simulink model "MMC_30_VSG_AD"  (R2023b)
settings: Solver=ode23t  StartTime=0.0  StopTime=2.4  RelTol=1e-3
InitFcn:
  | Rf=0.5929;
  | fn=50;
  | w0=2*pi*fn;
  | Lf=0.5*0.0135+0.01358;
  | R=0.5;
  | kf=8.5;
  | 
  | Kd=1.40543e+07;
  | lam=10; z0=0.707; zmax=1; wn0=lam/z0;
  | J0=223.613; DS0=4472.27;
  | Jmin=0.3*J0; Jmax=2.0*J0; Dmin=0.3*DS0; Dmax=2.2*DS0;
  | muJ=2906.97;
  | nu=0.15; nb=0.55; dzr=0.5; dzd=0;
  | tau=0.02; db=0.02; kpsi=14; txi=0.04;
  | Ts=0.0002; qref=0.03; dfref=0.064; dwref=0.4; dref=4;
  | lam_floor=1; scheme=1;
  | delta0=0.0712129;
  | J=J0; D=DS0;
libraries: spsIGBTDiodeLib x264, spsSeriesRLCBranchLib x140, spsVoltageMeasurementLib x132, spsCurrentMeasurementLib x6, spsSecondOrderFilterLib x3, spsThreePhaseVIMeasurementLib x2, spsDCVoltageSourceLib x2, slpidlib x2, spsGroundLib x1, spsPower3phInstantaneousLib x1, spsThreePhaseProgrammableVoltageSourceLib x1, spsThreePhaseSeriesRLCBranchLib x1
(part 5 of 5)

== system MMC_30_VSG_AD/MMC_INVERTER/MMC桥臂6/MMC子模块12 ==
  PWM : Inport
  IGBT/Diode : spsIGBTDiodeLib/IGBT//Diode  Ron=1e-3  Rs=1e5  Cs=inf  Measurements=off
  IGBT/Diode1 : spsIGBTDiodeLib/IGBT//Diode  Ron=1e-3  Rs=1e5  Cs=inf  Measurements=off
  Logical Operator : Logic  Inputs=1  AllPortsSameDT=off  OutDataTypeStr=boolean
  Logical Operator1 : Logic  Operator=NOT  AllPortsSameDT=off  OutDataTypeStr=boolean
  Series RLC Branch : spsSeriesRLCBranchLib/Series RLC Branch  LConnTagsString=__new0  RConnTagsString=__new0  BranchType=C  Resistance=1  Inductance=1e-3  SetiL0=off  InitialCurrent=0  Capacitance=C0  Setx0=on  InitialVoltage=V0  Measurements=None
  Voltage Measurement : spsVoltageMeasurementLib/Voltage Measurement  PhasorSimulation=off  OutputType=Complex  PSBequivalent=0
  V+ : PMIOPort  Side=Left
  V- : PMIOPort  Port=2  Side=Left
  VC : Outport
  wires:
  Logical Operator1/1 -> IGBT/Diode1/1
  Logical Operator/1 -> IGBT/Diode/1
  Voltage Measurement/1 -> VC/1
  PWM/1 -> Logical Operator/1, Logical Operator1/1
  connections:
  Voltage Measurement/LConn1 -- Series RLC Branch/LConn1 -- IGBT/Diode/LConn1
  V+/RConn1 -- IGBT/Diode/RConn1 -- IGBT/Diode1/LConn1
  V-/RConn1 -- IGBT/Diode1/RConn1 -- Series RLC Branch/RConn1 -- Voltage Measurement/LConn2

== system MMC_30_VSG_AD/MMC_INVERTER/MMC桥臂6/MMC子模块13 ==
  PWM : Inport
  IGBT/Diode : spsIGBTDiodeLib/IGBT//Diode  Ron=1e-3  Rs=1e5  Cs=inf  Measurements=off
  IGBT/Diode1 : spsIGBTDiodeLib/IGBT//Diode  Ron=1e-3  Rs=1e5  Cs=inf  Measurements=off
  Logical Operator : Logic  Inputs=1  AllPortsSameDT=off  OutDataTypeStr=boolean
  Logical Operator1 : Logic  Operator=NOT  AllPortsSameDT=off  OutDataTypeStr=boolean
  Series RLC Branch : spsSeriesRLCBranchLib/Series RLC Branch  LConnTagsString=__new0  RConnTagsString=__new0  BranchType=C  Resistance=1  Inductance=1e-3  SetiL0=off  InitialCurrent=0  Capacitance=C0  Setx0=on  InitialVoltage=V0  Measurements=None
  Voltage Measurement : spsVoltageMeasurementLib/Voltage Measurement  PhasorSimulation=off  OutputType=Complex  PSBequivalent=0
  V+ : PMIOPort  Side=Left
  V- : PMIOPort  Port=2  Side=Left
  VC : Outport
  wires:
  Logical Operator1/1 -> IGBT/Diode1/1
  Logical Operator/1 -> IGBT/Diode/1
  Voltage Measurement/1 -> VC/1
  PWM/1 -> Logical Operator/1, Logical Operator1/1
  connections:
  Voltage Measurement/LConn1 -- Series RLC Branch/LConn1 -- IGBT/Diode/LConn1
  V+/RConn1 -- IGBT/Diode/RConn1 -- IGBT/Diode1/LConn1
  V-/RConn1 -- IGBT/Diode1/RConn1 -- Series RLC Branch/RConn1 -- Voltage Measurement/LConn2

== system MMC_30_VSG_AD/MMC_INVERTER/MMC桥臂6/MMC子模块14 ==
  PWM : Inport
  IGBT/Diode : spsIGBTDiodeLib/IGBT//Diode  Ron=1e-3  Rs=1e5  Cs=inf  Measurements=off
  IGBT/Diode1 : spsIGBTDiodeLib/IGBT//Diode  Ron=1e-3  Rs=1e5  Cs=inf  Measurements=off
  Logical Operator : Logic  Inputs=1  AllPortsSameDT=off  OutDataTypeStr=boolean
  Logical Operator1 : Logic  Operator=NOT  AllPortsSameDT=off  OutDataTypeStr=boolean
  Series RLC Branch : spsSeriesRLCBranchLib/Series RLC Branch  LConnTagsString=__new0  RConnTagsString=__new0  BranchType=C  Resistance=1  Inductance=1e-3  SetiL0=off  InitialCurrent=0  Capacitance=C0  Setx0=on  InitialVoltage=V0  Measurements=None
  Voltage Measurement : spsVoltageMeasurementLib/Voltage Measurement  PhasorSimulation=off  OutputType=Complex  PSBequivalent=0
  V+ : PMIOPort  Side=Left
  V- : PMIOPort  Port=2  Side=Left
  VC : Outport
  wires:
  Logical Operator1/1 -> IGBT/Diode1/1
  Logical Operator/1 -> IGBT/Diode/1
  Voltage Measurement/1 -> VC/1
  PWM/1 -> Logical Operator/1, Logical Operator1/1
  connections:
  Voltage Measurement/LConn1 -- Series RLC Branch/LConn1 -- IGBT/Diode/LConn1
  V+/RConn1 -- IGBT/Diode/RConn1 -- IGBT/Diode1/LConn1
  V-/RConn1 -- IGBT/Diode1/RConn1 -- Series RLC Branch/RConn1 -- Voltage Measurement/LConn2

== system MMC_30_VSG_AD/MMC_INVERTER/MMC桥臂6/MMC子模块15 ==
  PWM : Inport
  IGBT/Diode : spsIGBTDiodeLib/IGBT//Diode  Ron=1e-3  Rs=1e5  Cs=inf  Measurements=off
  IGBT/Diode1 : spsIGBTDiodeLib/IGBT//Diode  Ron=1e-3  Rs=1e5  Cs=inf  Measurements=off
  Logical Operator : Logic  Inputs=1  AllPortsSameDT=off  OutDataTypeStr=boolean
  Logical Operator1 : Logic  Operator=NOT  AllPortsSameDT=off  OutDataTypeStr=boolean
  Series RLC Branch : spsSeriesRLCBranchLib/Series RLC Branch  LConnTagsString=__new0  RConnTagsString=__new0  BranchType=C  Resistance=1  Inductance=1e-3  SetiL0=off  InitialCurrent=0  Capacitance=C0  Setx0=on  InitialVoltage=V0  Measurements=None
  Voltage Measurement : spsVoltageMeasurementLib/Voltage Measurement  PhasorSimulation=off  OutputType=Complex  PSBequivalent=0
  V+ : PMIOPort  Side=Left
  V- : PMIOPort  Port=2  Side=Left
  VC : Outport
  wires:
  Logical Operator1/1 -> IGBT/Diode1/1
  Logical Operator/1 -> IGBT/Diode/1
  Voltage Measurement/1 -> VC/1
  PWM/1 -> Logical Operator/1, Logical Operator1/1
  connections:
  Voltage Measurement/LConn1 -- Series RLC Branch/LConn1 -- IGBT/Diode/LConn1
  V+/RConn1 -- IGBT/Diode/RConn1 -- IGBT/Diode1/LConn1
  V-/RConn1 -- IGBT/Diode1/RConn1 -- Series RLC Branch/RConn1 -- Voltage Measurement/LConn2

== system MMC_30_VSG_AD/MMC_INVERTER/MMC桥臂6/MMC子模块16 ==
  PWM : Inport
  IGBT/Diode : spsIGBTDiodeLib/IGBT//Diode  Ron=1e-3  Rs=1e5  Cs=inf  Measurements=off
  IGBT/Diode1 : spsIGBTDiodeLib/IGBT//Diode  Ron=1e-3  Rs=1e5  Cs=inf  Measurements=off
  Logical Operator : Logic  Inputs=1  AllPortsSameDT=off  OutDataTypeStr=boolean
  Logical Operator1 : Logic  Operator=NOT  AllPortsSameDT=off  OutDataTypeStr=boolean
  Series RLC Branch : spsSeriesRLCBranchLib/Series RLC Branch  LConnTagsString=__new0  RConnTagsString=__new0  BranchType=C  Resistance=1  Inductance=1e-3  SetiL0=off  InitialCurrent=0  Capacitance=C0  Setx0=on  InitialVoltage=V0  Measurements=None
  Voltage Measurement : spsVoltageMeasurementLib/Voltage Measurement  PhasorSimulation=off  OutputType=Complex  PSBequivalent=0
  V+ : PMIOPort  Side=Left
  V- : PMIOPort  Port=2  Side=Left
  VC : Outport
  wires:
  Logical Operator1/1 -> IGBT/Diode1/1
  Logical Operator/1 -> IGBT/Diode/1
  Voltage Measurement/1 -> VC/1
  PWM/1 -> Logical Operator/1, Logical Operator1/1
  connections:
  Voltage Measurement/LConn1 -- Series RLC Branch/LConn1 -- IGBT/Diode/LConn1
  V+/RConn1 -- IGBT/Diode/RConn1 -- IGBT/Diode1/LConn1
  V-/RConn1 -- IGBT/Diode1/RConn1 -- Series RLC Branch/RConn1 -- Voltage Measurement/LConn2

== system MMC_30_VSG_AD/MMC_INVERTER/MMC桥臂6/MMC子模块17 ==
  PWM : Inport
  IGBT/Diode : spsIGBTDiodeLib/IGBT//Diode  Ron=1e-3  Rs=1e5  Cs=inf  Measurements=off
  IGBT/Diode1 : spsIGBTDiodeLib/IGBT//Diode  Ron=1e-3  Rs=1e5  Cs=inf  Measurements=off
  Logical Operator : Logic  Inputs=1  AllPortsSameDT=off  OutDataTypeStr=boolean
  Logical Operator1 : Logic  Operator=NOT  AllPortsSameDT=off  OutDataTypeStr=boolean
  Series RLC Branch : spsSeriesRLCBranchLib/Series RLC Branch  LConnTagsString=__new0  RConnTagsString=__new0  BranchType=C  Resistance=1  Inductance=1e-3  SetiL0=off  InitialCurrent=0  Capacitance=C0  Setx0=on  InitialVoltage=V0  Measurements=None
  Voltage Measurement : spsVoltageMeasurementLib/Voltage Measurement  PhasorSimulation=off  OutputType=Complex  PSBequivalent=0
  V+ : PMIOPort  Side=Left
  V- : PMIOPort  Port=2  Side=Left
  VC : Outport
  wires:
  Logical Operator1/1 -> IGBT/Diode1/1
  Logical Operator/1 -> IGBT/Diode/1
  Voltage Measurement/1 -> VC/1
  PWM/1 -> Logical Operator/1, Logical Operator1/1
  connections:
  Voltage Measurement/LConn1 -- Series RLC Branch/LConn1 -- IGBT/Diode/LConn1
  V+/RConn1 -- IGBT/Diode/RConn1 -- IGBT/Diode1/LConn1
  V-/RConn1 -- IGBT/Diode1/RConn1 -- Series RLC Branch/RConn1 -- Voltage Measurement/LConn2

== system MMC_30_VSG_AD/MMC_INVERTER/MMC桥臂6/MMC子模块18 ==
  PWM : Inport
  IGBT/Diode : spsIGBTDiodeLib/IGBT//Diode  Ron=1e-3  Rs=1e5  Cs=inf  Measurements=off
  IGBT/Diode1 : spsIGBTDiodeLib/IGBT//Diode  Ron=1e-3  Rs=1e5  Cs=inf  Measurements=off
  Logical Operator : Logic  Inputs=1  AllPortsSameDT=off  OutDataTypeStr=boolean
  Logical Operator1 : Logic  Operator=NOT  AllPortsSameDT=off  OutDataTypeStr=boolean
  Series RLC Branch : spsSeriesRLCBranchLib/Series RLC Branch  LConnTagsString=__new0  RConnTagsString=__new0  BranchType=C  Resistance=1  Inductance=1e-3  SetiL0=off  InitialCurrent=0  Capacitance=C0  Setx0=on  InitialVoltage=V0  Measurements=None
  Voltage Measurement : spsVoltageMeasurementLib/Voltage Measurement  PhasorSimulation=off  OutputType=Complex  PSBequivalent=0
  V+ : PMIOPort  Side=Left
  V- : PMIOPort  Port=2  Side=Left
  VC : Outport
  wires:
  Logical Operator1/1 -> IGBT/Diode1/1
  Logical Operator/1 -> IGBT/Diode/1
  Voltage Measurement/1 -> VC/1
  PWM/1 -> Logical Operator/1, Logical Operator1/1
  connections:
  Voltage Measurement/LConn1 -- Series RLC Branch/LConn1 -- IGBT/Diode/LConn1
  V+/RConn1 -- IGBT/Diode/RConn1 -- IGBT/Diode1/LConn1
  V-/RConn1 -- IGBT/Diode1/RConn1 -- Series RLC Branch/RConn1 -- Voltage Measurement/LConn2

== system MMC_30_VSG_AD/MMC_INVERTER/MMC桥臂6/MMC子模块19 ==
  PWM : Inport
  IGBT/Diode : spsIGBTDiodeLib/IGBT//Diode  Ron=1e-3  Rs=1e5  Cs=inf  Measurements=off
  IGBT/Diode1 : spsIGBTDiodeLib/IGBT//Diode  Ron=1e-3  Rs=1e5  Cs=inf  Measurements=off
  Logical Operator : Logic  Inputs=1  AllPortsSameDT=off  OutDataTypeStr=boolean
  Logical Operator1 : Logic  Operator=NOT  AllPortsSameDT=off  OutDataTypeStr=boolean
  Series RLC Branch : spsSeriesRLCBranchLib/Series RLC Branch  LConnTagsString=__new0  RConnTagsString=__new0  BranchType=C  Resistance=1  Inductance=1e-3  SetiL0=off  InitialCurrent=0  Capacitance=C0  Setx0=on  InitialVoltage=V0  Measurements=None
  Voltage Measurement : spsVoltageMeasurementLib/Voltage Measurement  PhasorSimulation=off  OutputType=Complex  PSBequivalent=0
  V+ : PMIOPort  Side=Left
  V- : PMIOPort  Port=2  Side=Left
  VC : Outport
  wires:
  Logical Operator1/1 -> IGBT/Diode1/1
  Logical Operator/1 -> IGBT/Diode/1
  Voltage Measurement/1 -> VC/1
  PWM/1 -> Logical Operator/1, Logical Operator1/1
  connections:
  Voltage Measurement/LConn1 -- Series RLC Branch/LConn1 -- IGBT/Diode/LConn1
  V+/RConn1 -- IGBT/Diode/RConn1 -- IGBT/Diode1/LConn1
  V-/RConn1 -- IGBT/Diode1/RConn1 -- Series RLC Branch/RConn1 -- Voltage Measurement/LConn2

== system MMC_30_VSG_AD/MMC_INVERTER/MMC桥臂6/MMC子模块2 ==
  PWM : Inport
  IGBT/Diode : spsIGBTDiodeLib/IGBT//Diode  Ron=1e-3  Rs=1e5  Cs=inf  Measurements=off
  IGBT/Diode1 : spsIGBTDiodeLib/IGBT//Diode  Ron=1e-3  Rs=1e5  Cs=inf  Measurements=off
  Logical Operator : Logic  Inputs=1  AllPortsSameDT=off  OutDataTypeStr=boolean
  Logical Operator1 : Logic  Operator=NOT  AllPortsSameDT=off  OutDataTypeStr=boolean
  Series RLC Branch : spsSeriesRLCBranchLib/Series RLC Branch  LConnTagsString=__new0  RConnTagsString=__new0  BranchType=C  Resistance=1  Inductance=1e-3  SetiL0=off  InitialCurrent=0  Capacitance=C0  Setx0=on  InitialVoltage=V0  Measurements=None
  Voltage Measurement : spsVoltageMeasurementLib/Voltage Measurement  PhasorSimulation=off  OutputType=Complex  PSBequivalent=0
  V+ : PMIOPort  Side=Left
  V- : PMIOPort  Port=2  Side=Left
  VC : Outport
  wires:
  Logical Operator1/1 -> IGBT/Diode1/1
  Logical Operator/1 -> IGBT/Diode/1
  Voltage Measurement/1 -> VC/1
  PWM/1 -> Logical Operator/1, Logical Operator1/1
  connections:
  Voltage Measurement/LConn1 -- Series RLC Branch/LConn1 -- IGBT/Diode/LConn1
  V+/RConn1 -- IGBT/Diode/RConn1 -- IGBT/Diode1/LConn1
  V-/RConn1 -- IGBT/Diode1/RConn1 -- Series RLC Branch/RConn1 -- Voltage Measurement/LConn2

== system MMC_30_VSG_AD/MMC_INVERTER/MMC桥臂6/MMC子模块20 ==
  PWM : Inport
  IGBT/Diode : spsIGBTDiodeLib/IGBT//Diode  Ron=1e-3  Rs=1e5  Cs=inf  Measurements=off
  IGBT/Diode1 : spsIGBTDiodeLib/IGBT//Diode  Ron=1e-3  Rs=1e5  Cs=inf  Measurements=off
  Logical Operator : Logic  Inputs=1  AllPortsSameDT=off  OutDataTypeStr=boolean
  Logical Operator1 : Logic  Operator=NOT  AllPortsSameDT=off  OutDataTypeStr=boolean
  Series RLC Branch : spsSeriesRLCBranchLib/Series RLC Branch  LConnTagsString=__new0  RConnTagsString=__new0  BranchType=C  Resistance=1  Inductance=1e-3  SetiL0=off  InitialCurrent=0  Capacitance=C0  Setx0=on  InitialVoltage=V0  Measurements=None
  Voltage Measurement : spsVoltageMeasurementLib/Voltage Measurement  PhasorSimulation=off  OutputType=Complex  PSBequivalent=0
  V+ : PMIOPort  Side=Left
  V- : PMIOPort  Port=2  Side=Left
  VC : Outport
  wires:
  Logical Operator1/1 -> IGBT/Diode1/1
  Logical Operator/1 -> IGBT/Diode/1
  Voltage Measurement/1 -> VC/1
  PWM/1 -> Logical Operator/1, Logical Operator1/1
  connections:
  Voltage Measurement/LConn1 -- Series RLC Branch/LConn1 -- IGBT/Diode/LConn1
  V+/RConn1 -- IGBT/Diode/RConn1 -- IGBT/Diode1/LConn1
  V-/RConn1 -- IGBT/Diode1/RConn1 -- Series RLC Branch/RConn1 -- Voltage Measurement/LConn2

== system MMC_30_VSG_AD/MMC_INVERTER/MMC桥臂6/MMC子模块21 ==
  PWM : Inport
  IGBT/Diode : spsIGBTDiodeLib/IGBT//Diode  Ron=1e-3  Rs=1e5  Cs=inf  Measurements=off
  IGBT/Diode1 : spsIGBTDiodeLib/IGBT//Diode  Ron=1e-3  Rs=1e5  Cs=inf  Measurements=off
  Logical Operator : Logic  Inputs=1  AllPortsSameDT=off  OutDataTypeStr=boolean
  Logical Operator1 : Logic  Operator=NOT  AllPortsSameDT=off  OutDataTypeStr=boolean
  Series RLC Branch : spsSeriesRLCBranchLib/Series RLC Branch  LConnTagsString=__new0  RConnTagsString=__new0  BranchType=C  Resistance=1  Inductance=1e-3  SetiL0=off  InitialCurrent=0  Capacitance=C0  Setx0=on  InitialVoltage=V0  Measurements=None
  Voltage Measurement : spsVoltageMeasurementLib/Voltage Measurement  PhasorSimulation=off  OutputType=Complex  PSBequivalent=0
  V+ : PMIOPort  Side=Left
  V- : PMIOPort  Port=2  Side=Left
  VC : Outport
  wires:
  Logical Operator1/1 -> IGBT/Diode1/1
  Logical Operator/1 -> IGBT/Diode/1
  Voltage Measurement/1 -> VC/1
  PWM/1 -> Logical Operator/1, Logical Operator1/1
  connections:
  Voltage Measurement/LConn1 -- Series RLC Branch/LConn1 -- IGBT/Diode/LConn1
  V+/RConn1 -- IGBT/Diode/RConn1 -- IGBT/Diode1/LConn1
  V-/RConn1 -- IGBT/Diode1/RConn1 -- Series RLC Branch/RConn1 -- Voltage Measurement/LConn2

== system MMC_30_VSG_AD/MMC_INVERTER/MMC桥臂6/MMC子模块3 ==
  PWM : Inport
  IGBT/Diode : spsIGBTDiodeLib/IGBT//Diode  Ron=1e-3  Rs=1e5  Cs=inf  Measurements=off
  IGBT/Diode1 : spsIGBTDiodeLib/IGBT//Diode  Ron=1e-3  Rs=1e5  Cs=inf  Measurements=off
  Logical Operator : Logic  Inputs=1  AllPortsSameDT=off  OutDataTypeStr=boolean
  Logical Operator1 : Logic  Operator=NOT  AllPortsSameDT=off  OutDataTypeStr=boolean
  Series RLC Branch : spsSeriesRLCBranchLib/Series RLC Branch  LConnTagsString=__new0  RConnTagsString=__new0  BranchType=C  Resistance=1  Inductance=1e-3  SetiL0=off  InitialCurrent=0  Capacitance=C0  Setx0=on  InitialVoltage=V0  Measurements=None
  Voltage Measurement : spsVoltageMeasurementLib/Voltage Measurement  PhasorSimulation=off  OutputType=Complex  PSBequivalent=0
  V+ : PMIOPort  Side=Left
  V- : PMIOPort  Port=2  Side=Left
  VC : Outport
  wires:
  Logical Operator1/1 -> IGBT/Diode1/1
  Logical Operator/1 -> IGBT/Diode/1
  Voltage Measurement/1 -> VC/1
  PWM/1 -> Logical Operator/1, Logical Operator1/1
  connections:
  Voltage Measurement/LConn1 -- Series RLC Branch/LConn1 -- IGBT/Diode/LConn1
  V+/RConn1 -- IGBT/Diode/RConn1 -- IGBT/Diode1/LConn1
  V-/RConn1 -- IGBT/Diode1/RConn1 -- Series RLC Branch/RConn1 -- Voltage Measurement/LConn2

== system MMC_30_VSG_AD/MMC_INVERTER/MMC桥臂6/MMC子模块4 ==
  PWM : Inport
  IGBT/Diode : spsIGBTDiodeLib/IGBT//Diode  Ron=1e-3  Rs=1e5  Cs=inf  Measurements=off
  IGBT/Diode1 : spsIGBTDiodeLib/IGBT//Diode  Ron=1e-3  Rs=1e5  Cs=inf  Measurements=off
  Logical Operator : Logic  Inputs=1  AllPortsSameDT=off  OutDataTypeStr=boolean
  Logical Operator1 : Logic  Operator=NOT  AllPortsSameDT=off  OutDataTypeStr=boolean
  Series RLC Branch : spsSeriesRLCBranchLib/Series RLC Branch  LConnTagsString=__new0  RConnTagsString=__new0  BranchType=C  Resistance=1  Inductance=1e-3  SetiL0=off  InitialCurrent=0  Capacitance=C0  Setx0=on  InitialVoltage=V0  Measurements=None
  Voltage Measurement : spsVoltageMeasurementLib/Voltage Measurement  PhasorSimulation=off  OutputType=Complex  PSBequivalent=0
  V+ : PMIOPort  Side=Left
  V- : PMIOPort  Port=2  Side=Left
  VC : Outport
  wires:
  Logical Operator1/1 -> IGBT/Diode1/1
  Logical Operator/1 -> IGBT/Diode/1
  Voltage Measurement/1 -> VC/1
  PWM/1 -> Logical Operator/1, Logical Operator1/1
  connections:
  Voltage Measurement/LConn1 -- Series RLC Branch/LConn1 -- IGBT/Diode/LConn1
  V+/RConn1 -- IGBT/Diode/RConn1 -- IGBT/Diode1/LConn1
  V-/RConn1 -- IGBT/Diode1/RConn1 -- Series RLC Branch/RConn1 -- Voltage Measurement/LConn2

== system MMC_30_VSG_AD/MMC_INVERTER/MMC桥臂6/MMC子模块5 ==
  PWM : Inport
  IGBT/Diode : spsIGBTDiodeLib/IGBT//Diode  Ron=1e-3  Rs=1e5  Cs=inf  Measurements=off
  IGBT/Diode1 : spsIGBTDiodeLib/IGBT//Diode  Ron=1e-3  Rs=1e5  Cs=inf  Measurements=off
  Logical Operator : Logic  Inputs=1  AllPortsSameDT=off  OutDataTypeStr=boolean
  Logical Operator1 : Logic  Operator=NOT  AllPortsSameDT=off  OutDataTypeStr=boolean
  Series RLC Branch : spsSeriesRLCBranchLib/Series RLC Branch  LConnTagsString=__new0  RConnTagsString=__new0  BranchType=C  Resistance=1  Inductance=1e-3  SetiL0=off  InitialCurrent=0  Capacitance=C0  Setx0=on  InitialVoltage=V0  Measurements=None
  Voltage Measurement : spsVoltageMeasurementLib/Voltage Measurement  PhasorSimulation=off  OutputType=Complex  PSBequivalent=0
  V+ : PMIOPort  Side=Left
  V- : PMIOPort  Port=2  Side=Left
  VC : Outport
  wires:
  Logical Operator1/1 -> IGBT/Diode1/1
  Logical Operator/1 -> IGBT/Diode/1
  Voltage Measurement/1 -> VC/1
  PWM/1 -> Logical Operator/1, Logical Operator1/1
  connections:
  Voltage Measurement/LConn1 -- Series RLC Branch/LConn1 -- IGBT/Diode/LConn1
  V+/RConn1 -- IGBT/Diode/RConn1 -- IGBT/Diode1/LConn1
  V-/RConn1 -- IGBT/Diode1/RConn1 -- Series RLC Branch/RConn1 -- Voltage Measurement/LConn2

== system MMC_30_VSG_AD/MMC_INVERTER/MMC桥臂6/MMC子模块6 ==
  PWM : Inport
  IGBT/Diode : spsIGBTDiodeLib/IGBT//Diode  Ron=1e-3  Rs=1e5  Cs=inf  Measurements=off
  IGBT/Diode1 : spsIGBTDiodeLib/IGBT//Diode  Ron=1e-3  Rs=1e5  Cs=inf  Measurements=off
  Logical Operator : Logic  Inputs=1  AllPortsSameDT=off  OutDataTypeStr=boolean
  Logical Operator1 : Logic  Operator=NOT  AllPortsSameDT=off  OutDataTypeStr=boolean
  Series RLC Branch : spsSeriesRLCBranchLib/Series RLC Branch  LConnTagsString=__new0  RConnTagsString=__new0  BranchType=C  Resistance=1  Inductance=1e-3  SetiL0=off  InitialCurrent=0  Capacitance=C0  Setx0=on  InitialVoltage=V0  Measurements=None
  Voltage Measurement : spsVoltageMeasurementLib/Voltage Measurement  PhasorSimulation=off  OutputType=Complex  PSBequivalent=0
  V+ : PMIOPort  Side=Left
  V- : PMIOPort  Port=2  Side=Left
  VC : Outport
  wires:
  Logical Operator1/1 -> IGBT/Diode1/1
  Logical Operator/1 -> IGBT/Diode/1
  Voltage Measurement/1 -> VC/1
  PWM/1 -> Logical Operator/1, Logical Operator1/1
  connections:
  Voltage Measurement/LConn1 -- Series RLC Branch/LConn1 -- IGBT/Diode/LConn1
  V+/RConn1 -- IGBT/Diode/RConn1 -- IGBT/Diode1/LConn1
  V-/RConn1 -- IGBT/Diode1/RConn1 -- Series RLC Branch/RConn1 -- Voltage Measurement/LConn2

== system MMC_30_VSG_AD/MMC_INVERTER/MMC桥臂6/MMC子模块7 ==
  PWM : Inport
  IGBT/Diode : spsIGBTDiodeLib/IGBT//Diode  Ron=1e-3  Rs=1e5  Cs=inf  Measurements=off
  IGBT/Diode1 : spsIGBTDiodeLib/IGBT//Diode  Ron=1e-3  Rs=1e5  Cs=inf  Measurements=off
  Logical Operator : Logic  Inputs=1  AllPortsSameDT=off  OutDataTypeStr=boolean
  Logical Operator1 : Logic  Operator=NOT  AllPortsSameDT=off  OutDataTypeStr=boolean
  Series RLC Branch : spsSeriesRLCBranchLib/Series RLC Branch  LConnTagsString=__new0  RConnTagsString=__new0  BranchType=C  Resistance=1  Inductance=1e-3  SetiL0=off  InitialCurrent=0  Capacitance=C0  Setx0=on  InitialVoltage=V0  Measurements=None
  Voltage Measurement : spsVoltageMeasurementLib/Voltage Measurement  PhasorSimulation=off  OutputType=Complex  PSBequivalent=0
  V+ : PMIOPort  Side=Left
  V- : PMIOPort  Port=2  Side=Left
  VC : Outport
  wires:
  Logical Operator1/1 -> IGBT/Diode1/1
  Logical Operator/1 -> IGBT/Diode/1
  Voltage Measurement/1 -> VC/1
  PWM/1 -> Logical Operator/1, Logical Operator1/1
  connections:
  Voltage Measurement/LConn1 -- Series RLC Branch/LConn1 -- IGBT/Diode/LConn1
  V+/RConn1 -- IGBT/Diode/RConn1 -- IGBT/Diode1/LConn1
  V-/RConn1 -- IGBT/Diode1/RConn1 -- Series RLC Branch/RConn1 -- Voltage Measurement/LConn2

== system MMC_30_VSG_AD/MMC_INVERTER/MMC桥臂6/MMC子模块8 ==
  PWM : Inport
  IGBT/Diode : spsIGBTDiodeLib/IGBT//Diode  Ron=1e-3  Rs=1e5  Cs=inf  Measurements=off
  IGBT/Diode1 : spsIGBTDiodeLib/IGBT//Diode  Ron=1e-3  Rs=1e5  Cs=inf  Measurements=off
  Logical Operator : Logic  Inputs=1  AllPortsSameDT=off  OutDataTypeStr=boolean
  Logical Operator1 : Logic  Operator=NOT  AllPortsSameDT=off  OutDataTypeStr=boolean
  Series RLC Branch : spsSeriesRLCBranchLib/Series RLC Branch  LConnTagsString=__new0  RConnTagsString=__new0  BranchType=C  Resistance=1  Inductance=1e-3  SetiL0=off  InitialCurrent=0  Capacitance=C0  Setx0=on  InitialVoltage=V0  Measurements=None
  Voltage Measurement : spsVoltageMeasurementLib/Voltage Measurement  PhasorSimulation=off  OutputType=Complex  PSBequivalent=0
  V+ : PMIOPort  Side=Left
  V- : PMIOPort  Port=2  Side=Left
  VC : Outport
  wires:
  Logical Operator1/1 -> IGBT/Diode1/1
  Logical Operator/1 -> IGBT/Diode/1
  Voltage Measurement/1 -> VC/1
  PWM/1 -> Logical Operator/1, Logical Operator1/1
  connections:
  Voltage Measurement/LConn1 -- Series RLC Branch/LConn1 -- IGBT/Diode/LConn1
  V+/RConn1 -- IGBT/Diode/RConn1 -- IGBT/Diode1/LConn1
  V-/RConn1 -- IGBT/Diode1/RConn1 -- Series RLC Branch/RConn1 -- Voltage Measurement/LConn2

== system MMC_30_VSG_AD/MMC_INVERTER/MMC桥臂6/MMC子模块9 ==
  PWM : Inport
  IGBT/Diode : spsIGBTDiodeLib/IGBT//Diode  Ron=1e-3  Rs=1e5  Cs=inf  Measurements=off
  IGBT/Diode1 : spsIGBTDiodeLib/IGBT//Diode  Ron=1e-3  Rs=1e5  Cs=inf  Measurements=off
  Logical Operator : Logic  Inputs=1  AllPortsSameDT=off  OutDataTypeStr=boolean
  Logical Operator1 : Logic  Operator=NOT  AllPortsSameDT=off  OutDataTypeStr=boolean
  Series RLC Branch : spsSeriesRLCBranchLib/Series RLC Branch  LConnTagsString=__new0  RConnTagsString=__new0  BranchType=C  Resistance=1  Inductance=1e-3  SetiL0=off  InitialCurrent=0  Capacitance=C0  Setx0=on  InitialVoltage=V0  Measurements=None
  Voltage Measurement : spsVoltageMeasurementLib/Voltage Measurement  PhasorSimulation=off  OutputType=Complex  PSBequivalent=0
  V+ : PMIOPort  Side=Left
  V- : PMIOPort  Port=2  Side=Left
  VC : Outport
  wires:
  Logical Operator1/1 -> IGBT/Diode1/1
  Logical Operator/1 -> IGBT/Diode/1
  Voltage Measurement/1 -> VC/1
  PWM/1 -> Logical Operator/1, Logical Operator1/1
  connections:
  Voltage Measurement/LConn1 -- Series RLC Branch/LConn1 -- IGBT/Diode/LConn1
  V+/RConn1 -- IGBT/Diode/RConn1 -- IGBT/Diode1/LConn1
  V-/RConn1 -- IGBT/Diode1/RConn1 -- Series RLC Branch/RConn1 -- Voltage Measurement/LConn2

== matlab function MMC_30_VSG_AD/VSG控制/VSG有功控制-频率调节-一次调频/adap_law ==
  data: dw input; Jm output; Dm output; wn_o output; z_o output; xi_o output; Ts parameter; tau parameter; qref parameter; txi parameter; kpsi parameter; db parameter; wn0 parameter; nu parameter; nb parameter; z0 parameter; dzd parameter; dzr parameter; lam parameter; zmax parameter; Kd parameter; lam_floor parameter; scheme parameter; Jmin parameter; Jmax parameter; Dmin parameter; Dmax parameter; w0 parameter
function [Jm, Dm, wn_o, z_o, xi_o] = adap_law(dw, Ts, tau, qref, txi, kpsi, db, wn0, nu, nb, z0, dzd, dzr, lam, zmax, Kd, lam_floor, scheme, Jmin, Jmax, Dmin, Dmax, w0)





persistent dwf dwp ddwf xf first


if isempty(first)


    dwf = 0; dwp = 0; ddwf = 0; xf = 0; first = 1;


end


a = Ts/(tau + Ts);


dwf = dwf + a*(dw - dwf);               


d1  = (dwf - dwp)/Ts;


dwp = dwf;


ddwf = ddwf + a*(d1 - ddwf);             


xi = dwf*ddwf/max(qref, 1e-9);


if txi > 0


    xf = xf + (xi - xf)*Ts/txi;          


    xi = xf;


end


s  = (2/pi)*atan(kpsi*(xi - db*tanh(xi/db)));  


sp = max(s, 0);


sm = min(s, 0);


wn = wn0*(1 - nu*sp - nb*sm);


zs = z0 + dzd*sp - dzr*sm;


if lam_floor > 0


    zf = lam/wn;


else


    zf = z0;


end


z = min(max(max(zs, zf), z0), zmax);


Jp = Kd/wn^2;


Dp = 2*z*sqrt(Kd*Jp);


switch scheme


    case 1


        Jp = Kd/wn0^2;  Dp = 2*z0*sqrt(Kd*Jp);


    otherwise


end


Jm = Jp/w0;


Dm = Dp/w0;


Jm = min(max(Jm, Jmin), Jmax);


Dm = min(max(Dm, Dmin), Dmax);


wn_o = wn;  z_o = z;  xi_o = xi;


end

== matlab function MMC_30_VSG_AD/电流环控制器/MATLAB Function2 ==
  data: d input; a output; q input; wt input; b output; c output
function [a,b,c] = dqtoabc(d,q,wt)
a=cos(wt)*d-sin(wt)*q;
b=cos(wt-2*pi/3)*d-sin(wt-2*pi/3)*q;
c=cos(wt+2*pi/3)*d-sin(wt+2*pi/3)*q;

== matlab function MMC_30_VSG_AD/最近电平逼近NLM/NLM ==
  data: VA input; VAP output; VB input; VC input; VAL output; HLA input; HLB input; HLC input; VBP output; VBL output; VCP output; VCL output; VDC input; V1 input
function [VAP,VAL,VBP,VBL,VCP,VCL] = NLM(VA,VB,VC,HLA,HLB,HLC, VDC, V1)
%初始值
% VDC=11000;
% V1=500;
%最近电平逼近
VAP=VDC/(2*V1)-round((VA+HLA)/V1);
VAL=VDC/(2*V1)+round((VA-HLA)/V1);
VBP=VDC/(2*V1)-round((VB+HLB)/V1);
VBL=VDC/(2*V1)+round((VB-HLB)/V1);
VCP=VDC/(2*V1)-round((VC+HLC)/V1);
VCL=VDC/(2*V1)+round((VC-HLC)/V1);

== matlab function MMC_30_VSG_AD/PWM波输出/均压程序 ==
  settings: updateMethod=DISCRETE
  data: VP input; PWM_P output; VL input; ip input; PWM_L output; il input; V_p input; V_low input; Ts input
function [PWM_P,PWM_L] = JY(VP,VL,ip,il,V_p,V_low,Ts)
%初始化
persistent pwm_p pwm_low
k=22;
if isempty(pwm_p)
    pwm_p=zeros(k,1);
    pwm_low=zeros(k,1);
end
%满足条件进入
if(Ts==0)
    a=k;
    P=zeros(2,k);
    L=zeros(2,k);
    %输入电容替换
    for i=1:a
        P(1,i)=V_p(i);
        P(2,i)=i;
        L(1,i)=V_low(i);
        L(2,i)=i;
    end
    %冒泡排序
    for i=1:a-1
        for j=1:a-i
            if P(1,j)>P(1,j+1)
                t1=P(1,j);
                t2=P(2,j);
                P(1,j)=P(1,j+1);
                P(2,j)=P(2,j+1);
                P(1,j+1)=t1;
                P(2,j+1)=t2;
            end
            if L(1,j)>L(1,j+1)
                t1=L(1,j);
                t2=L(2,j);
                L(1,j)=L(1,j+1);
                L(2,j)=L(2,j+1);
                L(1,j+1)=t1;
                L(2,j+1)=t2;
            end
        end
    end
    pwm_p=zeros(k,1);
    pwm_low=zeros(k,1);
    %判断桥臂电流方向，确定电容充放电
    %上桥臂电流方向
    if VP<=0
        pwm_p=zeros(k,1);
    elseif VP<a
        if ip>0
            for i=1:VP
                pwm_p(P(2,i),1)=1;
            end
        else
            for i=a-VP+1:a
                pwm_p(P(2,i),1)=1;
            end
        end
    else
        pwm_p=ones(k,1);
    end
    %下桥臂电流方向
    if VL<=0
        pwm_low=zeros(k,1);
    elseif VL<a
        if il>0
            for i=1:VL
                pwm_low(L(2,i),1)=1;
            end
        else
            for i=a-VL+1:a
                pwm_low(L(2,i),1)=1;
            end
        end
    else
        pwm_low=ones(k,1);
    end
end
PWM_P=pwm_p;
PWM_L=pwm_low;

== matlab function MMC_30_VSG_AD/PWM波输出/均压程序2 ==
  settings: updateMethod=DISCRETE
  data: VP input; PWM_P output; VL input; ip input; PWM_L output; il input; V_p input; V_low input; Ts input
function [PWM_P,PWM_L] = JY(VP,VL,ip,il,V_p,V_low,Ts)
%初始化
persistent pwm_p pwm_low
k=22;
if isempty(pwm_p)
    pwm_p=zeros(k,1);
    pwm_low=zeros(k,1);
end
%满足条件进入
if(Ts==0)
    a=k;
    P=zeros(2,k);
    L=zeros(2,k);
    %输入电容替换
    for i=1:a
        P(1,i)=V_p(i);
        P(2,i)=i;
        L(1,i)=V_low(i);
        L(2,i)=i;
    end
    %冒泡排序
    for i=1:a-1
        for j=1:a-i
            if P(1,j)>P(1,j+1)
                t1=P(1,j);
                t2=P(2,j);
                P(1,j)=P(1,j+1);
                P(2,j)=P(2,j+1);
                P(1,j+1)=t1;
                P(2,j+1)=t2;
            end
            if L(1,j)>L(1,j+1)
                t1=L(1,j);
                t2=L(2,j);
                L(1,j)=L(1,j+1);
                L(2,j)=L(2,j+1);
                L(1,j+1)=t1;
                L(2,j+1)=t2;
            end
        end
    end
    pwm_p=zeros(k,1);
    pwm_low=zeros(k,1);
    %判断桥臂电流方向，确定电容充放电
    %上桥臂电流方向
    if VP<=0
        pwm_p=zeros(k,1);
    elseif VP<a
        if ip>0
            for i=1:VP
                pwm_p(P(2,i),1)=1;
            end
        else
            for i=a-VP+1:a
                pwm_p(P(2,i),1)=1;
            end
        end
    else
        pwm_p=ones(k,1);
    end
    %下桥臂电流方向
    if VL<=0
        pwm_low=zeros(k,1);
    elseif VL<a
        if il>0
            for i=1:VL
                pwm_low(L(2,i),1)=1;
            end
        else
            for i=a-VL+1:a
                pwm_low(L(2,i),1)=1;
            end
        end
    else
        pwm_low=ones(k,1);
    end
end
PWM_P=pwm_p;
PWM_L=pwm_low;

== matlab function MMC_30_VSG_AD/PWM波输出/均压程序3 ==
  settings: updateMethod=DISCRETE
  data: VP input; PWM_P output; VL input; ip input; PWM_L output; il input; V_p input; V_low input; Ts input
function [PWM_P,PWM_L] = JY(VP,VL,ip,il,V_p,V_low,Ts)
%初始化
persistent pwm_p pwm_low
k=22;
if isempty(pwm_p)
    pwm_p=zeros(k,1);
    pwm_low=zeros(k,1);
end
%满足条件进入
if(Ts==0)
    a=k;
    P=zeros(2,k);
    L=zeros(2,k);
    %输入电容替换
    for i=1:a
        P(1,i)=V_p(i);
        P(2,i)=i;
        L(1,i)=V_low(i);
        L(2,i)=i;
    end
    %冒泡排序
    for i=1:a-1
        for j=1:a-i
            if P(1,j)>P(1,j+1)
                t1=P(1,j);
                t2=P(2,j);
                P(1,j)=P(1,j+1);
                P(2,j)=P(2,j+1);
                P(1,j+1)=t1;
                P(2,j+1)=t2;
            end
            if L(1,j)>L(1,j+1)
                t1=L(1,j);
                t2=L(2,j);
                L(1,j)=L(1,j+1);
                L(2,j)=L(2,j+1);
                L(1,j+1)=t1;
                L(2,j+1)=t2;
            end
        end
    end
    pwm_p=zeros(k,1);
    pwm_low=zeros(k,1);
    %判断桥臂电流方向，确定电容充放电
    %上桥臂电流方向
    if VP<=0
        pwm_p=zeros(k,1);
    elseif VP<a
        if ip>0
            for i=1:VP
                pwm_p(P(2,i),1)=1;
            end
        else
            for i=a-VP+1:a
                pwm_p(P(2,i),1)=1;
            end
        end
    else
        pwm_p=ones(k,1);
    end
    %下桥臂电流方向
    if VL<=0
        pwm_low=zeros(k,1);
    elseif VL<a
        if il>0
            for i=1:VL
                pwm_low(L(2,i),1)=1;
            end
        else
            for i=a-VL+1:a
                pwm_low(L(2,i),1)=1;
            end
        end
    else
        pwm_low=ones(k,1);
    end
end
PWM_P=pwm_p;
PWM_L=pwm_low;

== matlab function MMC_30_VSG_AD/abc-dq/MATLAB Function ==
  data: a input; alpha output; b input; c input; beta output
function [alpha,beta] = abctoalphabeta(a,b,c)
alpha=(2/3)*(a-b/2-c/2);
beta=(2/3)*((sqrt(3)/2)*(b-c));

== matlab function MMC_30_VSG_AD/abc-dq/MATLAB Function1 ==
  data: alpha input; d output; beta input; wt input; q output
function [d,q] = alphabetatodq(alpha,beta,wt)
d=cos(wt)*alpha+sin(wt)*beta;
q=-sin(wt)*alpha+cos(wt)*beta;

== matlab function MMC_30_VSG_AD/坐标变换1/abctoalpha//beta ==
  settings: updateMethod=DISCRETE
  data: a input; alpha output; b input; c input; beta output
function [alpha,beta] = abctoalphabeta(a,b,c)
alpha=(2/3)*(a-b/2-c/2);
beta=(2/3)*((sqrt(3)/2)*(b-c));

== matlab function MMC_30_VSG_AD/坐标变换1/abctoalpha//beta1 ==
  settings: updateMethod=DISCRETE
  data: a input; alpha output; b input; c input; beta output
function [alpha,beta] = abctoalphabeta(a,b,c)
alpha=(2/3)*(a-b/2-c/2);
beta=(2/3)*((sqrt(3)/2)*(b-c));

== matlab function MMC_30_VSG_AD/坐标变换1/dq ==
  settings: updateMethod=DISCRETE
  data: alpha input; d output; beta input; wt input; q output
function [d,q] = alphabetatodq(alpha,beta,wt)
d=cos(wt)*alpha+sin(wt)*beta;
q=-sin(wt)*alpha+cos(wt)*beta;

== matlab function MMC_30_VSG_AD/坐标变换1/dq1 ==
  settings: updateMethod=DISCRETE
  data: alpha input; d output; beta input; wt input; q output
function [d,q] = alphabetatodq(alpha,beta,wt)
d=cos(wt)*alpha+sin(wt)*beta;
q=-sin(wt)*alpha+cos(wt)*beta;
